simulink model "dpc_same_input_comparison"  (R2022a)
settings: Solver=FixedStepDiscrete  StartTime=0  StopTime=dpc_replay_stop  FixedStep=dpc_replay_cfg.sample_time  RelTol=1e-3
undefined symbols (not defined in the file): dpc_replay_cfg
Description:
  | Structurally authored comparison graph; rebuild natively via build_dpc_replay_model. No Simulink execution claimed.
settings SolverCC: AlgebraicLoopSolver=TrustRegion
settings DataIOCC: SaveOutput=off  SignalLogging=off  SaveTime=off
settings OptimizationCC: LifeSpan=inf
settings DebuggingCC: UnconnectedInputMsg=warning  UnconnectedOutputMsg=warning  UnconnectedLineMsg=warning  SFMachineParentedDataDiag=warning  ArithmeticOperatorsInVariantConditions=warning
settings SFSimCC: SimUseLocalCustomCode=off  CustomCodeUndefinedFunction=UseInterfaceOnly
settings RTWCC: RTWUseLocalCustomCode=off  DLArmComputeVersion=19.05
settings CodeAppCC: StateflowObjectComments=on

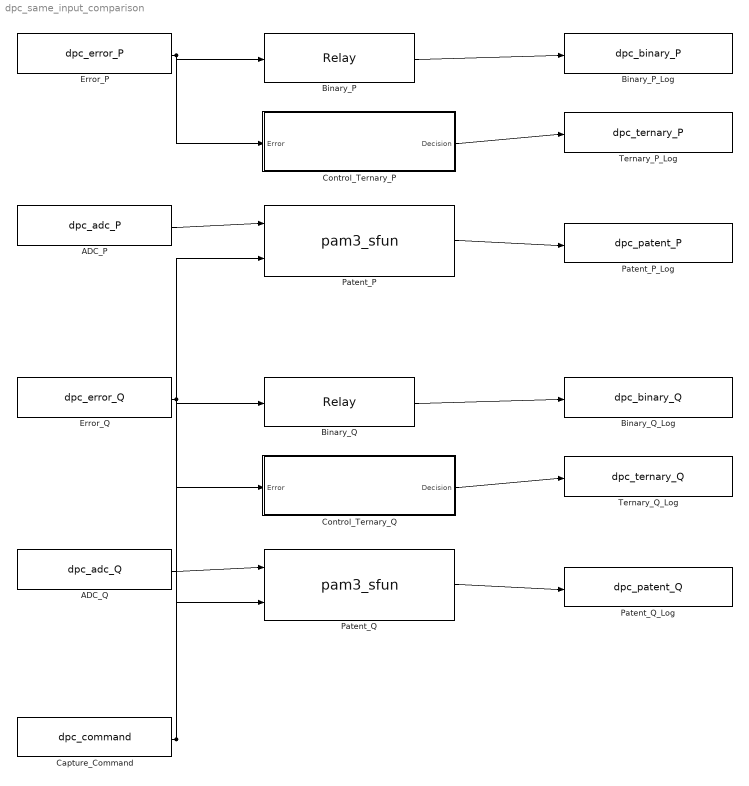
== system dpc_same_input_comparison ==
  Error_P : FromWorkspace  VariableName=dpc_error_P  SampleTime=dpc_replay_cfg.sample_time  Interpolate=off  OutputAfterFinalValue=Holding final value
  ADC_P : FromWorkspace  VariableName=dpc_adc_P  SampleTime=dpc_replay_cfg.sample_time  Interpolate=off  OutputAfterFinalValue=Holding final value
  Binary_P : Relay  OnSwitchValue=1  OffSwitchValue=-1  OnOutputValue=1  OffOutputValue=0  SampleTime=dpc_replay_cfg.sample_time
  Control_Ternary_P : Subsystem
  Patent_P : M-S-Function  FunctionName=pam3_sfun  Parameters=dpc_patent_cfg  DisplayMFileStacktrace=on
  Binary_P_Log : ToWorkspace  VariableName=dpc_binary_P  SaveFormat=Structure With Time  SampleTime=-1
  Ternary_P_Log : ToWorkspace  VariableName=dpc_ternary_P  SaveFormat=Structure With Time  SampleTime=-1
  Patent_P_Log : ToWorkspace  VariableName=dpc_patent_P  SaveFormat=Structure With Time  SampleTime=-1
  Error_Q : FromWorkspace  VariableName=dpc_error_Q  SampleTime=dpc_replay_cfg.sample_time  Interpolate=off  OutputAfterFinalValue=Holding final value
  ADC_Q : FromWorkspace  VariableName=dpc_adc_Q  SampleTime=dpc_replay_cfg.sample_time  Interpolate=off  OutputAfterFinalValue=Holding final value
  Binary_Q : Relay  OnSwitchValue=1  OffSwitchValue=-1  OnOutputValue=1  OffOutputValue=0  SampleTime=dpc_replay_cfg.sample_time
  Control_Ternary_Q : Subsystem
  Patent_Q : M-S-Function  FunctionName=pam3_sfun  Parameters=dpc_patent_cfg  DisplayMFileStacktrace=on
  Binary_Q_Log : ToWorkspace  VariableName=dpc_binary_Q  SaveFormat=Structure With Time  SampleTime=-1
  Ternary_Q_Log : ToWorkspace  VariableName=dpc_ternary_Q  SaveFormat=Structure With Time  SampleTime=-1
  Patent_Q_Log : ToWorkspace  VariableName=dpc_patent_Q  SaveFormat=Structure With Time  SampleTime=-1
  Capture_Command : FromWorkspace  VariableName=dpc_command  SampleTime=dpc_replay_cfg.sample_time  Interpolate=off  OutputAfterFinalValue=Holding final value
  wires:
  Error_P/1 -> Binary_P/1, Control_Ternary_P/1(Error)
  ADC_P/1 -> Patent_P/1
  Binary_P/1 -> Binary_P_Log/1
  Control_Ternary_P/1(Decision) -> Ternary_P_Log/1
  Patent_P/1 -> Patent_P_Log/1
  Error_Q/1 -> Binary_Q/1, Control_Ternary_Q/1(Error)
  ADC_Q/1 -> Patent_Q/1
  Binary_Q/1 -> Binary_Q_Log/1
  Control_Ternary_Q/1(Decision) -> Ternary_Q_Log/1
  Patent_Q/1 -> Patent_Q_Log/1
  Capture_Command/1 -> Patent_P/2, Patent_Q/2

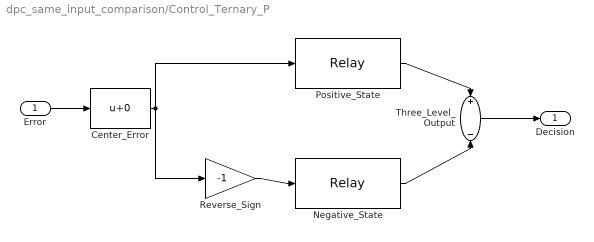
== system dpc_same_input_comparison/Control_Ternary_P ==
  Error : Inport  Port=1
  Center_Error : Bias  Bias=0
  Reverse_Sign : Gain  Gain=-1
  Positive_State : Relay  OnSwitchValue=1  OffSwitchValue=0.5  OnOutputValue=1  OffOutputValue=0  SampleTime=dpc_replay_cfg.sample_time
  Negative_State : Relay  OnSwitchValue=1  OffSwitchValue=0.5  OnOutputValue=1  OffOutputValue=0  SampleTime=dpc_replay_cfg.sample_time
  Three_Level_Output : Sum  Inputs=+-
  Decision : Outport  Port=1
  wires:
  Error/1 -> Center_Error/1
  Center_Error/1 -> Positive_State/1, Reverse_Sign/1
  Reverse_Sign/1 -> Negative_State/1
  Positive_State/1 -> Three_Level_Output/1
  Negative_State/1 -> Three_Level_Output/2
  Three_Level_Output/1 -> Decision/1

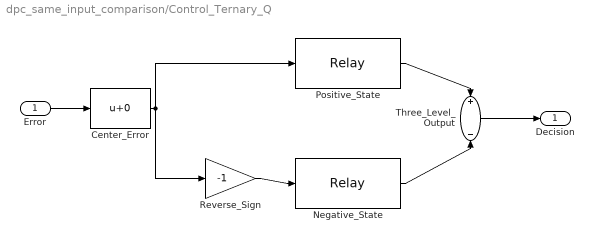
== system dpc_same_input_comparison/Control_Ternary_Q ==
  Error : Inport  Port=1
  Center_Error : Bias  Bias=0
  Reverse_Sign : Gain  Gain=-1
  Positive_State : Relay  OnSwitchValue=1  OffSwitchValue=0.5  OnOutputValue=1  OffOutputValue=0  SampleTime=dpc_replay_cfg.sample_time
  Negative_State : Relay  OnSwitchValue=1  OffSwitchValue=0.5  OnOutputValue=1  OffOutputValue=0  SampleTime=dpc_replay_cfg.sample_time
  Three_Level_Output : Sum  Inputs=+-
  Decision : Outport  Port=1
  wires:
  Error/1 -> Center_Error/1
  Center_Error/1 -> Positive_State/1, Reverse_Sign/1
  Reverse_Sign/1 -> Negative_State/1
  Positive_State/1 -> Three_Level_Output/1
  Negative_State/1 -> Three_Level_Output/2
  Three_Level_Output/1 -> Decision/1
